simulink model "can-signal-sim"  (R2024b)
settings: Solver=VariableStepAuto  StartTime=0.0  StopTime=inf  RelTol=1e-3
undefined symbols (not defined in the file): Blinktakt, canChannel, Normal
libraries: canlib x14, canmsglib x12, simulink x6
settings Model: Creator=MBade  LastModifiedBy=MBade

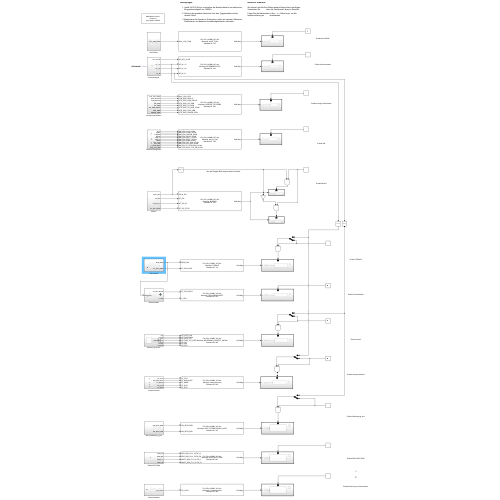
[thumbnail: Simulink's stored preview of the top-level diagram]
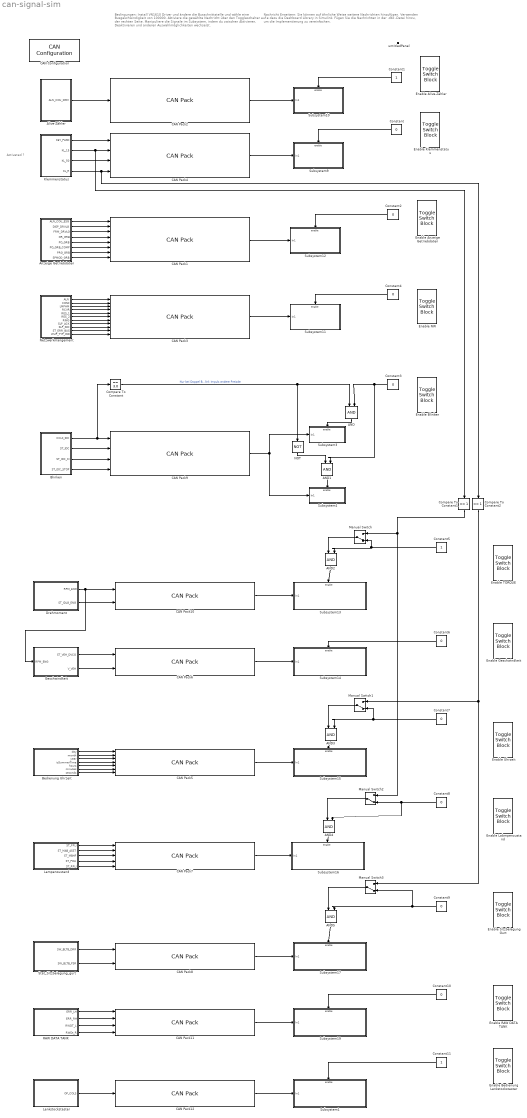
== system can-signal-sim ==
  note: Nachricht Erweitern:
      | Sie können auf ähnliche Weise weitere Nachrichten hinzufügen. Verwenden Sie dazu die Dashboard Library in Simulink.
      | Fügen Sie die Nachrichten in der .dbc -Datei hinzu, um die Implementierung zu vereinfachen.
  note: Bedingungen:
      | Install VN1610 Driver und ändere die Busschnittstelle und wähle eine Busgeschwindigkeit von 100000.
      | Aktiviere die gewählte Nachricht über den Toggleschalter auf der rechten Seite.
      | Manipuliere die Signale im Subsystem, indem du zwischen Aktivieren, Deaktivieren und anderen Auswahlmöglichkeiten wechselst.
  note: Activated ?
  AND{,1..5} (6 alike) : Logic  IconShape=distinctive  AllPortsSameDT=off  OutDataTypeStr=boolean
  Alive-Zähler : Subsystem
  Anzeige Getriebdaten : Subsystem
  Bedienung Uhrzeit : Subsystem
  Blinken : Subsystem
  CAN Configuration : canlib/CAN Configuration  BlockHandle=614.0004  Device=MathWorks Virtual 1 (Channel 1)  DeviceMenu=MathWorks Virtual 1 (Channel 1)  ObjConstructor=canChannel('MathWorks', 'Virtual 1', 1)  BusSpeed=100000  EnableBitParameters=off  AckMode=Normal
  CAN Pack1 : canmsglib/CAN Pack  CANdbFile=C:\Users\MBade\Desktop\GITHUB\Instrument-Cluster\PKW_Kombiinstruments\E9x_KOMBI_V07.dbc  MsgList=ANZEIGE_GETRIEBE  MsgName=ANZEIGE_GETRIEBE  MsgIDType=Standard (11-bit identifier)  MsgIdentifier=466  CANIDInput=off  MsgLength=6  Remote=off  ApplyMinMax=off  BusOutput=off  SignalInfo={'ALIV_COU_EGS','28','4','LE','unsigned','Standard','0','1','0','0','15';'CTR_DISP_DRVLG','40','4','LE','unsigned','Standard','0','1','0','0','15';'CTR_DISP_FRM_DRVLG','44','4','LE','unsigned','Standard','0','1','0','0','15';'CTR_DISP_GR_GRB','12','4','LE','unsigned','Standard','0','1','0','0','15';'CTR_DISP_PO_GRB','0','4','LE','unsigned','Standard','0','1','0','0','15';'CTR_DISP_PO_GRB_COMP','4','4','LE','unsigned','Standard','0','1','0','0','15';'CTR_DISP_PRG_GRB','32','4','LE','unsigned','Standard','0','1','0','0','15';'CTR_DISP_SPMOD_GRB','26','2','LE','unsigned','Standard','0','1','0','0','3'}
      settings: LibrarySourceBlock=canlib/CAN Pack  DataFormat=CANdb specified signals
  CAN Pack10 : canmsglib/CAN Pack  CANdbFile=C:\Users\MBade\MATLAB\Projects\PKW_Kombiinstruments\E9x_KOMBI_V07.dbc  MsgList=TORQUE  MsgName=TORQUE  MsgIDType=Standard (11-bit identifier)  MsgIdentifier=170  CANIDInput=off  MsgLength=8  Remote=off  ApplyMinMax=off  BusOutput=off  SignalInfo={'RPM_ENG','32','16','LE','unsigned','Standard','0','0.25','0','0','16383.75';'ST_IDLG_ENG','50','2','LE','unsigned','Standard','0','1','0','0','3'}
      settings: LibrarySourceBlock=canlib/CAN Pack  DataFormat=CANdb specified signals
  CAN Pack11 : canmsglib/CAN Pack  CANdbFile=C:\Users\MBade\MATLAB\Projects\PKW_Kombiinstruments\E9x_KOMBI_V07.dbc  MsgList=RAW_DATA_TANK  MsgName=RAW_DATA_TANK  MsgIDType=Standard (11-bit identifier)  MsgIdentifier=841  CANIDInput=off  MsgLength=5  Remote=off  ApplyMinMax=off  BusOutput=off  SignalInfo={'ERR_SEN_FLLV_FUTA_LH','32','4','LE','unsigned','Standard','0','1','0','0','15';'ERR_SEN_FLLV_FUTA_RH','36','4','LE','unsigned','Standard','0','1','0','0','15';'RWDT_SEN_FLLV_FUTA_L','0','16','LE','unsigned','Standard','0','0.1','0','0','6553.5';'RWDT_SEN_FLLV_FUTA_R','16','16','LE','unsigned','Standard','0','0.1','0','0','6553.5'}
      settings: LibrarySourceBlock=canlib/CAN Pack  DataFormat=CANdb specified signals
  CAN Pack12 : canmsglib/CAN Pack  CANdbFile=C:\Users\MBade\MATLAB\Projects\PKW_Kombiinstruments\E9x_KOMBI_V07.dbc  MsgList=Lenkstockstaster  MsgName=Lenkstockstaster  MsgIDType=Standard (11-bit identifier)  MsgIdentifier=494  CANIDInput=off  MsgLength=2  Remote=off  ApplyMinMax=off  BusOutput=off  SignalInfo={'OP_COLS','0','8','LE','unsigned','Standard','0','1','0','-Inf','Inf'}
      settings: LibrarySourceBlock=canlib/CAN Pack  DataFormat=CANdb specified signals
  CAN Pack2 : canmsglib/CAN Pack  CANdbFile=C:\Users\MBade\Desktop\GITHUB\Instrument-Cluster\PKW_Kombiinstruments\E9x_KOMBI_V07.dbc  MsgList=ALIVE_ZGM  MsgName=ALIVE_ZGM  MsgIDType=Standard (11-bit identifier)  MsgIdentifier=192  CANIDInput=off  MsgLength=2  Remote=off  ApplyMinMax=off  BusOutput=off  SignalInfo={'ALIV_COU_ZGM','0','4','LE','unsigned','Standard','0','1','0','0','15'}
      settings: LibrarySourceBlock=canlib/CAN Pack  DataFormat=CANdb specified signals
  CAN Pack3 : canmsglib/CAN Pack  CANdbFile=C:\Users\MBade\Desktop\GITHUB\Instrument-Cluster\PKW_Kombiinstruments\E9x_KOMBI_V07.dbc  MsgList=NM_K_CAN  MsgName=NM_K_CAN  MsgIDType=Standard (11-bit identifier)  MsgIdentifier=1152  CANIDInput=off  MsgLength=8  Remote=off  ApplyMinMax=off  BusOutput=off  SignalInfo={'NM_PDU_ALIV_KCAN','8','1','LE','unsigned','Standard','0','1','0','0','1';'NM_PDU_CONF_KCAN','14','1','LE','unsigned','Standard','0','1','0','0','1';'NM_PDU_LMPHM_KCAN','10','1','LE','unsigned','Standard','0','1','0','0','1';'NM_PDU_RCVR_KCAN','0','8','LE','unsigned','Standard','0','1','0','0','255';'NM_PDU_RES_1_KCAN','11','1','LE','unsigned','Standard','0','1','0','0','1';'NM_PDU_RES_2_KCAN','15','1','LE','unsigned','Standard','0','1','0','0','1';'NM_PDU_RING_KCAN','9','1','LE','unsigned','Standard','0','1','0','0','1';'NM_PDU_SLP_ACK_KCAN','13','1','LE','unsigned','Standard','0','1','0','0','1';'NM_PDU_SLP_IND_KCAN','12','1','LE','unsigned','Standard','0','1','0','0','1';'NM_PDU_ST_ERR_BUS_KCAN','24','8','LE','unsigned','Standard','0','1','0','0','255';'NM_PDU_WUP_TYP_IND_KCAN','16','2','LE','unsigned','Standard','0','1','0','0','3'}
      settings: LibrarySourceBlock=canlib/CAN Pack  DataFormat=CANdb specified signals
  CAN Pack4 : canmsglib/CAN Pack  CANdbFile=C:\Users\MBade\Desktop\GITHUB\Instrument-Cluster\PKW_Kombiinstruments\E9x_KOMBI_V07.dbc  MsgList=KLEMMENSTATUS  MsgName=KLEMMENSTATUS  MsgIDType=Standard (11-bit identifier)  MsgIdentifier=304  CANIDInput=off  MsgLength=5  Remote=off  ApplyMinMax=off  BusOutput=off  SignalInfo={'ST_KEY_PLGD','16','2','LE','unsigned','Standard','0','1','0','0','3';'ST_KL_15','2','2','LE','unsigned','Standard','0','1','0','0','3';'ST_KL_50','4','2','LE','unsigned','Standard','0','1','0','0','3';'ST_KL_R','0','2','LE','unsigned','Standard','0','1','0','0','3'}
      settings: LibrarySourceBlock=canlib/CAN Pack  DataFormat=CANdb specified signals
  CAN Pack5 : canmsglib/CAN Pack  CANdbFile=C:\Users\MBade\MATLAB\Projects\PKW_Kombiinstruments\E9x_KOMBI_V07.dbc  MsgList=BEDIENUNG_UHRZEIT_DATUM  MsgName=BEDIENUNG_UHRZEIT_DATUM  MsgIDType=Standard (11-bit identifier)  MsgIdentifier=926  CANIDInput=off  MsgLength=8  Remote=off  ApplyMinMax=off  BusOutput=off  SignalInfo={'OP_DATE_DAY','24','8','LE','unsigned','Standard','0','1','0','0','255';'OP_DATE_MON','36','4','LE','unsigned','Standard','0','1','0','0','15';'OP_DATE_YR','40','16','LE','unsigned','Standard','0','1','0','0','65535';'OP_DISP_CTI_DATE','56','4','LE','unsigned','Standard','0','1','0','0','15';'OP_HR','0','8','LE','unsigned','Standard','0','1','0','0','255';'OP_MN','8','8','LE','unsigned','Standard','0','1','0','0','255';'OP_SEC','16','8','LE','unsigned','Standard','0','1','0','0','255'}
      settings: LibrarySourceBlock=canlib/CAN Pack  DataFormat=CANdb specified signals
  CAN Pack6 : canmsglib/CAN Pack  CANdbFile=C:\Users\MBade\MATLAB\Projects\PKW_Kombiinstruments\E9x_KOMBI_V07.dbc  MsgList=GESCHWINDIGKEIT  MsgName=GESCHWINDIGKEIT  MsgIDType=Standard (11-bit identifier)  MsgIdentifier=416  CANIDInput=off  MsgLength=8  Remote=off  ApplyMinMax=off  BusOutput=off  SignalInfo={'ST_VEH_DVCO','12','3','LE','unsigned','Standard','0','1','0','0','7';'V_VEH','0','12','LE','unsigned','Standard','0','0.1','0','0','409.5'}
      settings: LibrarySourceBlock=canlib/CAN Pack  DataFormat=CANdb specified signals
  CAN Pack7 : canmsglib/CAN Pack  CANdbFile=C:\Users\MBade\MATLAB\Projects\PKW_Kombiinstruments\E9x_KOMBI_V07.dbc  MsgList=Lampenzustand  MsgName=Lampenzustand  MsgIDType=Standard (11-bit identifier)  MsgIdentifier=538  CANIDInput=off  MsgLength=3  Remote=off  ApplyMinMax=off  BusOutput=off  SignalInfo={'ST_FFLI','5','1','LE','unsigned','Standard','0','1','0','-Inf','Inf';'ST_MAB_ASST','18','2','LE','unsigned','Standard','0','1','0','-Inf','Inf';'ST_MBHF','1','1','LE','unsigned','Standard','0','1','0','-Inf','Inf';'ST_POLI','2','1','LE','unsigned','Standard','0','1','0','-Inf','Inf';'ST_RFLI','6','1','LE','unsigned','Standard','0','1','0','-Inf','Inf'}
      settings: LibrarySourceBlock=canlib/CAN Pack  DataFormat=CANdb specified signals
  CAN Pack8 : canmsglib/CAN Pack  CANdbFile=C:\Users\MBade\MATLAB\Projects\PKW_Kombiinstruments\E9x_KOMBI_V07.dbc  MsgList=STAT_SITZBELEGUNG_GURT  MsgName=STAT_SITZBELEGUNG_GURT  MsgIDType=Standard (11-bit identifier)  MsgIdentifier=762  CANIDInput=off  MsgLength=5  Remote=off  ApplyMinMax=off  BusOutput=off  SignalInfo={'SW_BLTB_DRR','28','2','LE','unsigned','Standard','0','1','0','0','3';'SW_BLTB_PSR','30','2','LE','unsigned','Standard','0','1','0','0','3'}
      settings: LibrarySourceBlock=canlib/CAN Pack  DataFormat=CANdb specified signals
  CAN Pack9 : canmsglib/CAN Pack  CANdbFile=C:\Users\MBade\MATLAB\Projects\PKW_Kombiinstruments\E9x_KOMBI_V07.dbc  MsgList=BLINKEN  MsgName=BLINKEN  MsgIDType=Standard (11-bit identifier)  MsgIdentifier=502  CANIDInput=off  MsgLength=2  Remote=off  ApplyMinMax=off  BusOutput=off  SignalInfo={'CCLK_IDC','0','4','LE','unsigned','Standard','0','1','0','0','15';'ST_IDC','4','3','LE','unsigned','Standard','0','1','0','0','7';'ST_IDC_KI','10','2','LE','unsigned','Standard','0','1','0','0','3';'ST_IDC_STOP','8','2','LE','unsigned','Standard','0','1','0','0','3'}
      settings: LibrarySourceBlock=canlib/CAN Pack  DataFormat=CANdb specified signals
  Compare To Constant : simulink/Logic and Bit Operations/Compare To Constant  relop===  const=3.0  OutDataTypeStr=boolean
  Compare To Constant1 : simulink/Logic and Bit Operations/Compare To Constant  relop===  const=1  OutDataTypeStr=boolean
  Compare To Constant2 : simulink/Logic and Bit Operations/Compare To Constant  relop===  const=1  OutDataTypeStr=boolean
  Constant{,2..4,6..10} (9 alike) : Constant  Value=0
  Constant1 : Constant
  Constant11 : Constant
  Constant5 : Constant
  Drehmoment : Subsystem
  Enable Alive-Zähler : ToggleSwitchBlock
      settings: Values={{'Off', 'On'}, [0 1]}
  Enable Anzeige Getriebdaten : ToggleSwitchBlock
      settings: Values={{'Off', 'On'}, [0 1]}
  Enable Bedienung Lenkstockstaster : ToggleSwitchBlock
      settings: Values={{'Off', 'On'}, [0 1]}
  Enable Blinken : ToggleSwitchBlock
      settings: Values={{'Off', 'On'}, [0 1]}
  Enable Geschwindkeit : ToggleSwitchBlock
      settings: Values={{'Off', 'On'}, [0 1]}
  Enable Klemmenstatus : ToggleSwitchBlock
      settings: Values={{'Off', 'On'}, [0 1]}
  Enable Labmpenzustand : ToggleSwitchBlock
      settings: Values={{'Off', 'On'}, [0 1]}
  Enable NW : ToggleSwitchBlock
      settings: Values={{'Off', 'On'}, [0 1]}
  Enable RAW DATA TANK : ToggleSwitchBlock
      settings: Values={{'Off', 'On'}, [0 1]}
  Enable Sitzbelegung Gurt : ToggleSwitchBlock
      settings: Values={{'Off', 'On'}, [0 1]}
  Enable TORQUE : ToggleSwitchBlock
      settings: Values={{'Off', 'On'}, [0 1]}
  Enable Uhrzeit : ToggleSwitchBlock
      settings: Values={{'Off', 'On'}, [0 1]}
  Geschwindkeit : Subsystem
  Klemmenstatus : Subsystem
  Lampenzustand : Subsystem
  Lenkstockstaster : Subsystem
  Manual Switch{,1..3} (4 alike) : ManualSwitch  CurrentSetting=0
  NOT : Logic  Operator=NOT  IconShape=distinctive  AllPortsSameDT=off  OutDataTypeStr=boolean
  Netzwerkmangement : Subsystem
  RAW DATA TANK : Subsystem
  Stat_Sitzbelegung_gurt : Subsystem
  Subsystem1 : Subsystem
  Subsystem10 : Subsystem
  Subsystem11 : Subsystem
  Subsystem12 : Subsystem
  Subsystem13 : Subsystem
  Subsystem14 : Subsystem
  Subsystem15 : Subsystem
  Subsystem16 : Subsystem
  Subsystem17 : Subsystem
  Subsystem19 : Subsystem
  Subsystem3 : Subsystem
  Subsystem4 : Subsystem
  Subsystem9 : Subsystem
  untitledPanel : Subsystem  Tag=HiddenForWebPanel  IsWebBlockPanel=on
  wires:
  Anzeige Getriebdaten/5(PO_GRB) -> CAN Pack1/5
  Anzeige Getriebdaten/6(PO_GRB_COMP) -> CAN Pack1/6
  Anzeige Getriebdaten/2(DISP_DRVLG) -> CAN Pack1/2
  Anzeige Getriebdaten/1(ALIV_COU_ESG) -> CAN Pack1/1
  Anzeige Getriebdaten/3(FRM_DRVLG) -> CAN Pack1/3
  Anzeige Getriebdaten/4(GR_GRB) -> CAN Pack1/4
  Anzeige Getriebdaten/8(SPMOD_GRB) -> CAN Pack1/8
  Anzeige Getriebdaten/7(PRG_GRB) -> CAN Pack1/7
  Alive-Zähler/1(ALIV_COU_ZGM) -> CAN Pack2/1
  Netzwerkmangement/5(RES_1) -> CAN Pack3/5
  Netzwerkmangement/7(RING) -> CAN Pack3/7
  Netzwerkmangement/6(RES_2) -> CAN Pack3/6
  Netzwerkmangement/4(RCVR) -> CAN Pack3/4
  Netzwerkmangement/8(SLP_ACK) -> CAN Pack3/8
  Netzwerkmangement/11(WUP_TYP_IND) -> CAN Pack3/11
  Netzwerkmangement/2(CONF) -> CAN Pack3/2
  Netzwerkmangement/9(SLP_IND) -> CAN Pack3/9
  Netzwerkmangement/10(ST_ERR_BUS) -> CAN Pack3/10
  Netzwerkmangement/1(ALIV) -> CAN Pack3/1
  Netzwerkmangement/3(LMPHM) -> CAN Pack3/3
  Klemmenstatus/1(KEY_PLGD) -> CAN Pack4/1
  Klemmenstatus/3(KL_50) -> CAN Pack4/3
  Klemmenstatus/4(KL_R) -> Compare To Constant2/1, CAN Pack4/4
  Blinken/1(CCLK_IDC) -> Compare To Constant/1, CAN Pack9/1
  Blinken/2(ST_IDC) -> CAN Pack9/2
  Blinken/3(ST_IDC_KI) -> CAN Pack9/3
  Blinken/4(ST_IDC_STOP) -> CAN Pack9/4
  Compare To Constant/1 -> AND/1, NOT/1  "Nur bei Doppel Blink Impuls andere Preiode"
  CAN Pack9/1 -> Subsystem4/1(In1), Subsystem3/1(In1)
  Drehmoment/1(RPM_ENG) -> CAN Pack10/1, Geschwindkeit/1(RPM_ENG)
  Drehmoment/2(ST_IDLG_ENG) -> CAN Pack10/2
  Geschwindkeit/1(ST_VEH_DVCO) -> CAN Pack6/1
  Geschwindkeit/2(V_VEH) -> CAN Pack6/2
  Klemmenstatus/2(KL_15) -> CAN Pack4/2, Compare To Constant1/1
  Compare To Constant1/1 -> Manual Switch2/1, Manual Switch/1
  Bedienung Uhrzeit/1(day) -> CAN Pack5/1
  Bedienung Uhrzeit/2(month) -> CAN Pack5/2
  Bedienung Uhrzeit/3(year) -> CAN Pack5/3
  Bedienung Uhrzeit/4(isSummerTime) -> CAN Pack5/4
  Bedienung Uhrzeit/5(hours) -> CAN Pack5/5
  Bedienung Uhrzeit/6(minutes) -> CAN Pack5/6
  Bedienung Uhrzeit/7(seconds) -> CAN Pack5/7
  Lampenzustand/1(ST_FFLI) -> CAN Pack7/1
  Lampenzustand/2(ST_MAB_ASST) -> CAN Pack7/2
  Lampenzustand/3(ST_MBHF) -> CAN Pack7/3
  Lampenzustand/4(ST_POLI) -> CAN Pack7/4
  Lampenzustand/5(ST_RFLI) -> CAN Pack7/5
  CAN Pack4/1 -> Subsystem9/1(In1)
  Constant/1 -> Subsystem9/Enable
  CAN Pack2/1 -> Subsystem10/1(In1)
  Constant1/1 -> Subsystem10/Enable
  CAN Pack3/1 -> Subsystem11/1(In1)
  CAN Pack1/1 -> Subsystem12/1(In1)
  Constant2/1 -> Subsystem12/Enable
  Constant4/1 -> Subsystem11/Enable
  NOT/1 -> AND1/1
  Constant3/1 -> AND/2, AND1/2
  AND1/1 -> Subsystem4/Enable
  AND/1 -> Subsystem3/Enable
  CAN Pack10/1 -> Subsystem13/1(In1)
  AND2/1 -> Subsystem13/Enable
  Constant5/1 -> AND2/2, Manual Switch/2
  Manual Switch/1 -> AND2/1
  CAN Pack6/1 -> Subsystem14/1(In1)
  Constant6/1 -> Subsystem14/Enable
  CAN Pack5/1 -> Subsystem15/1(In1)
  AND3/1 -> Subsystem15/Enable
  Constant7/1 -> AND3/2, Manual Switch1/2
  Compare To Constant2/1 -> Manual Switch1/1, Manual Switch3/1
  Manual Switch1/1 -> AND3/1
  CAN Pack7/1 -> Subsystem16/1(In1)
  AND4/1 -> Subsystem16/Enable
  Manual Switch2/1 -> AND4/1
  Constant8/1 -> Manual Switch2/2, AND4/2
  AND5/1 -> Subsystem17/Enable
  Manual Switch3/1 -> AND5/1
  Constant9/1 -> Manual Switch3/2, AND5/2
  CAN Pack8/1 -> Subsystem17/1(In1)
  Stat_Sitzbelegung_gurt/1(SW_BLTB_DRR) -> CAN Pack8/1
  Stat_Sitzbelegung_gurt/2(SW_BLTB_PSR) -> CAN Pack8/2
  CAN Pack11/1 -> Subsystem19/1(In1)
  Constant10/1 -> Subsystem19/Enable
  RAW DATA TANK/1(ERR_LH) -> CAN Pack11/1
  RAW DATA TANK/3(RWDT_L) -> CAN Pack11/3
  RAW DATA TANK/2(ERR_RH) -> CAN Pack11/2
  RAW DATA TANK/4(RWDt_R) -> CAN Pack11/4
  Constant11/1 -> Subsystem1/Enable
  CAN Pack12/1 -> Subsystem1/1(In1)
  Lenkstockstaster/1(OP_COLS) -> CAN Pack12/1

== system can-signal-sim/Alive-Zähler ==
  note: Die Versendung dieser Nachricht erfolgt zyklisch bei Bus aktiv.
  Constant : Constant  Value=15  OutDataTypeStr=uint8  SampleTime=0.2
  Counter Limited1 : simulink/Sources/Counter Limited  uplimit=14  tsamp=0.2
  Display : Display
      settings: Format=binary (Stored Integer)
  Manual Switch : ManualSwitch
  Scope : Scope
  ALIV_COU_ZGM : Outport
  wires:
  Manual Switch/1 -> Display/1, ALIV_COU_ZGM/1, Scope/1  "ALIV_COU_ZGM"
  Constant/1 -> Manual Switch/2  "Signal ungültig"
  Counter Limited1/1 -> Manual Switch/1

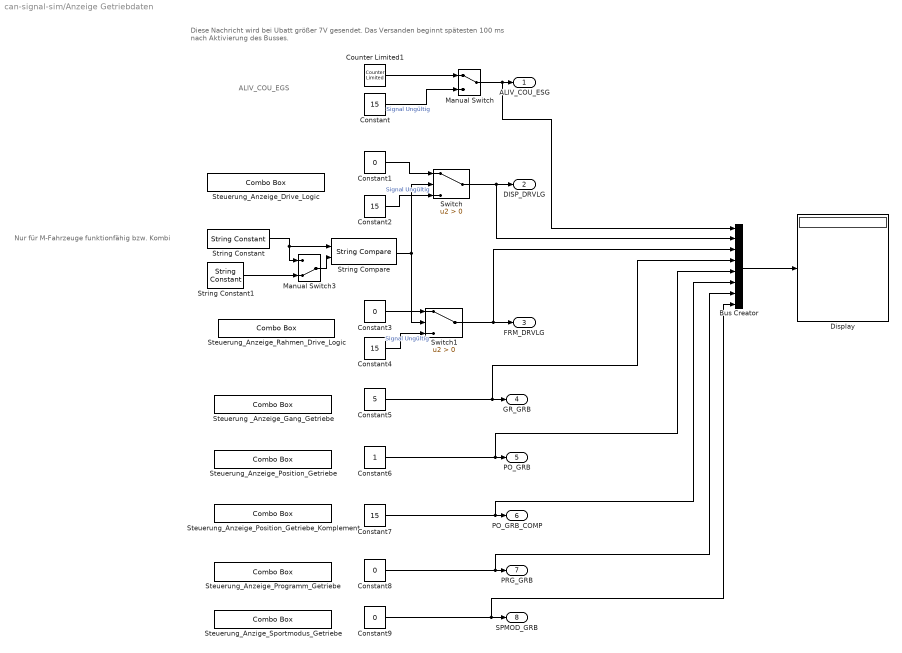
== system can-signal-sim/Anzeige Getriebdaten ==
  note: Nur für M-Fahrzeuge funktionfähig bzw. Kombi
  note: ALIV_COU_EGS
  note: Diese Nachricht wird bei Ubatt größer 7V gesendet. Das Versanden beginnt spätesten 100 ms nach Aktivierung des Busses.
  Bus Creator : BusCreator  Inputs=8
  Constant{,2,4,7} (4 alike) : Constant  Value=15  SampleTime=0.2
  Constant{1,3,8..9} (4 alike) : Constant  Value=0  SampleTime=0.2
  Constant5 : Constant  Value=5  SampleTime=0.2
  Constant6 : Constant  SampleTime=0.2
  Counter Limited1 : simulink/Sources/Counter Limited  uplimit=14  tsamp=0.2
  Display : Display
      settings: Format=binary (Stored Integer)
  Manual Switch : ManualSwitch
  Manual Switch3 : ManualSwitch  CurrentSetting=0
  Steuerung _Anzeige_Gang_Getriebe : ComboBox  LabelPosition=Hide  SelectedLabel=1.Gang
      settings: Values={{'Dunkelschaltung', '1.Gang', '2.Gang', '3.Gang', '4.Gang', '5.Gang', '6.Gang', '7.Gang', '8.Gang', 'Signal ungültig'}, [0 5 6 7 8 9 10 11 12 15]}
  Steuerung_Anzeige_Drive_Logic : ComboBox  LabelPosition=Hide  SelectedLabel=Dunkelschaltung
      settings: Values={{'Dunkelschaltung', '1', '2', '3', '4', '5', '6', 'Signal ungültig'}, [0 1 2 3 4 5 6 15]}
  Steuerung_Anzeige_Position_Getriebe : ComboBox  LabelPosition=Hide  SelectedLabel=P
      settings: Values={{'Dunkelschaltung', 'P', 'R', 'P_30sec', 'N', 'N_30,5min', 'N-5min', 'D', 'Signal ungültig'}, [0 1 2 3 4 6 7 8 15]}
  Steuerung_Anzeige_Position_Getriebe_Komplement : ComboBox  LabelPosition=Hide  SelectedLabel=Dunkelschaltung
      settings: Values={{'Dunkelschaltung', 'P', 'R', 'P_30sec', 'N', 'N_30,5min', 'N_5min', 'D', 'Signal ungültig'}, [15 14 13 12 11 9 8 7 0]}
  Steuerung_Anzeige_Programm_Getriebe : ComboBox  LabelPosition=Hide  SelectedLabel=Dunkelschaltung
      settings: Values={{'Dunkelschaltung', 'S-Programm', 'M-Programm', 'L-Programm', 'C-Programm', 'Signal ungültig'}, [0 1 2 4 8 15]}
  Steuerung_Anzeige_Rahmen_Drive_Logic : ComboBox  LabelPosition=Hide  SelectedLabel=Dunkelschaltung
      settings: Values={{'Dunkelschaltung', 'An, 5 Segmente', 'An, 6 Segmente', 'Signal ungültig'}, [0 5 6 15]}
  Steuerung_Anzige_Sportmodus_Getriebe : ComboBox  LabelPosition=Hide  SelectedLabel=Normalmodus
      settings: Values={{'Normalmodus', 'Sportmodus', 'Signal ungültig'}, [0 1 3]}
  String Compare : StringCompare
  String Constant : StringConstant  String="\"M_Fahrzeugen\""
  String Constant1 : StringConstant  String="\"anders\""
  Switch : Switch  Criteria=u2 > Threshold  SaturateOnIntegerOverflow=off  InputSameDT=off
  Switch1 : Switch  Criteria=u2 > Threshold  SaturateOnIntegerOverflow=off  InputSameDT=off
  ALIV_COU_ESG : Outport
  DISP_DRVLG : Outport  Port=2
  FRM_DRVLG : Outport  Port=3
  GR_GRB : Outport  Port=4
  PO_GRB : Outport  Port=5
  PO_GRB_COMP : Outport  Port=6
  PRG_GRB : Outport  Port=7
  SPMOD_GRB : Outport  Port=8
  wires:
  Counter Limited1/1 -> Manual Switch/1
  Manual Switch/1 -> ALIV_COU_ESG/1, Bus Creator/1
  Switch1/1 -> Bus Creator/3, FRM_DRVLG/1
  Constant/1 -> Manual Switch/2  "Signal Ungültig"
  Constant5/1 -> Bus Creator/4, GR_GRB/1
  Constant6/1 -> Bus Creator/5, PO_GRB/1
  Constant7/1 -> Bus Creator/6, PO_GRB_COMP/1
  Constant8/1 -> Bus Creator/7, PRG_GRB/1
  Constant9/1 -> Bus Creator/8, SPMOD_GRB/1
  String Constant/1 -> Manual Switch3/1, String Compare/1
  String Constant1/1 -> Manual Switch3/2
  Manual Switch3/1 -> String Compare/2
  String Compare/1 -> Switch/2, Switch1/2
  Constant1/1 -> Switch/1
  Constant2/1 -> Switch/3  "Signal Ungültig"
  Switch/1 -> Bus Creator/2, DISP_DRVLG/1
  Constant4/1 -> Switch1/3  "Signal Ungültig"
  Constant3/1 -> Switch1/1
  Bus Creator/1 -> Display/1

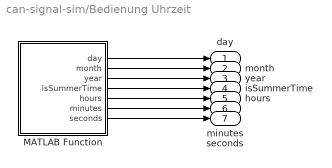
== system can-signal-sim/Bedienung Uhrzeit ==
  MATLAB Function : MATLAB Function  TreatAsAtomicUnit=on
  day : Outport
  month : Outport  Port=2
  year : Outport  Port=3
  isSummerTime : Outport  Port=4
  hours : Outport  Port=5
  minutes : Outport  Port=6
  seconds : Outport  Port=7
  wires:
  MATLAB Function/4(isSummerTime) -> isSummerTime/1
  MATLAB Function/6(minutes) -> minutes/1
  MATLAB Function/5(hours) -> hours/1
  MATLAB Function/7(seconds) -> seconds/1
  MATLAB Function/3(year) -> year/1
  MATLAB Function/2(month) -> month/1
  MATLAB Function/1(day) -> day/1

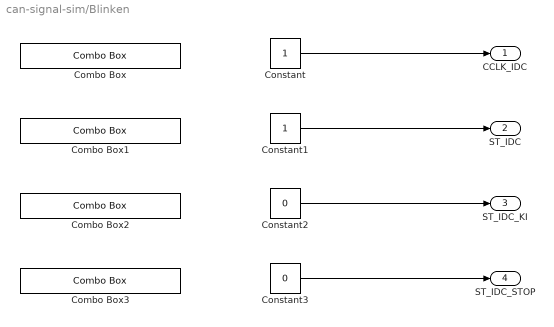
== system can-signal-sim/Blinken ==
  Combo Box : ComboBox  LabelPosition=Hide  SelectedLabel=Normal-Blinktakt
      settings: Values={{'Nicht blinken', 'Normal-Blinktakt', 'Defekt-Blinktakt', 'Doppel-Blink-Impuls', 'Signal ungültig'}, [0 1 2 3 15]}
  Combo Box1 : ComboBox  LabelPosition=Hide  SelectedLabel=Blinker link Ein
      settings: Values={{'Beide Blinker AUS', 'Blinker link Ein', 'Blinker rechts Ein', 'Beide Blinker Ein', 'Signal ungültig'}, [0 1 2 3 7]}
  Combo Box2 : ComboBox  LabelPosition=Hide  SelectedLabel=Blinktakt läuft weiter
      settings: Values={{'Blinktakt läuft weiter', 'Synchronisation', 'Neuen Blinktakt starten', 'Signal ungültig'}, [0 1 2 3]}
  Combo Box3 : ComboBox  LabelPosition=Hide  SelectedLabel=Blinkerkontroll-Lampen im Kombi signalisieren
      settings: Values={{'Blinkerkontroll-Lampen im Kombi signalisieren', 'Blinkerkontroll-Lampen im verdecktes Blinken', 'Signal ungültig'}, [0 1 3]}
  Constant : Constant
  Constant1 : Constant
  Constant2 : Constant  Value=0
  Constant3 : Constant  Value=0
  CCLK_IDC : Outport
  ST_IDC : Outport  Port=2
  ST_IDC_KI : Outport  Port=3
  ST_IDC_STOP : Outport  Port=4
  wires:
  Constant/1 -> CCLK_IDC/1
  Constant1/1 -> ST_IDC/1
  Constant2/1 -> ST_IDC_KI/1
  Constant3/1 -> ST_IDC_STOP/1

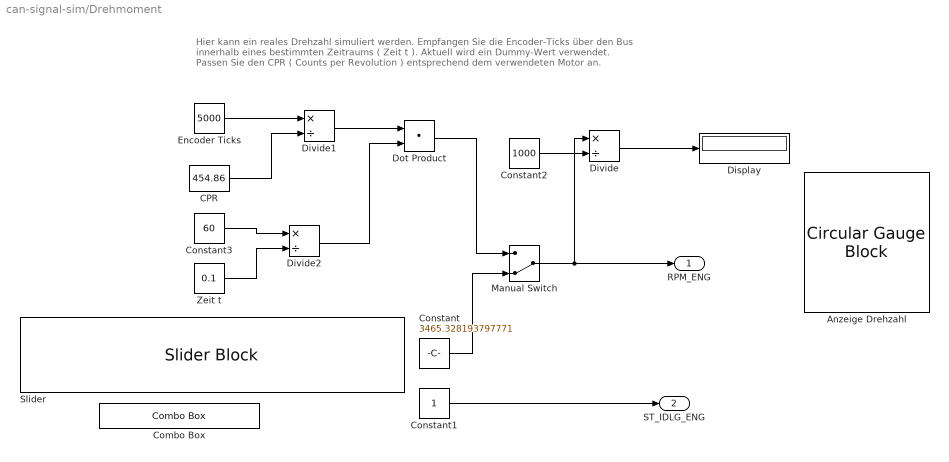
== system can-signal-sim/Drehmoment ==
  note: Hier kann ein reales Drehzahl simuliert werden.
      | Empfangen Sie die Encoder-Ticks über den Bus innerhalb eines bestimmten Zeitraums ( Zeit t ).
      | Aktuell wird ein Dummy-Wert verwendet.
      | Passen Sie den CPR ( Counts per Revolution ) entsprechend dem verwendeten Motor an.
  Anzeige Drehzahl : CircularGaugeBlock  ScaleMax=6  TickInterval=1
  CPR : Constant  Value=454.86
  Combo Box : ComboBox  LabelPosition=Hide  SelectedLabel=Motor nicht im Leerlauf
      settings: Values={{'Leerlauf', 'Motor nicht im Leerlauf', 'Label3'}, [0 1 3]}
  Constant : Constant  Value=3465.328193797771  OutMax=[16383.75]
  Constant1 : Constant
  Constant2 : Constant  Value=1000
  Constant3 : Constant  Value=60
  Display : Display
  Divide : Product  Inputs=*/
  Divide1 : Product  Inputs=*/
  Divide2 : Product  Inputs=*/
  Dot Product : DotProduct  OutDataTypeStr=Inherit: Inherit via internal rule
  Encoder Ticks : Constant  Value=5000
  Manual Switch : ManualSwitch  CurrentSetting=0
  Slider : SliderBlock  ScaleMax=16383.75
  Zeit t : Constant  Value=0.1
  RPM_ENG : Outport
  ST_IDLG_ENG : Outport  Port=2
  wires:
  Constant1/1 -> ST_IDLG_ENG/1
  Constant/1 -> Manual Switch/2
  Manual Switch/1 -> RPM_ENG/1, Divide/1
  Constant2/1 -> Divide/2
  Encoder Ticks/1 -> Divide1/1
  CPR/1 -> Divide1/2
  Constant3/1 -> Divide2/1
  Divide2/1 -> Dot Product/2
  Divide1/1 -> Dot Product/1
  Zeit t/1 -> Divide2/2
  Dot Product/1 -> Manual Switch/1
  Divide/1 -> Display/1

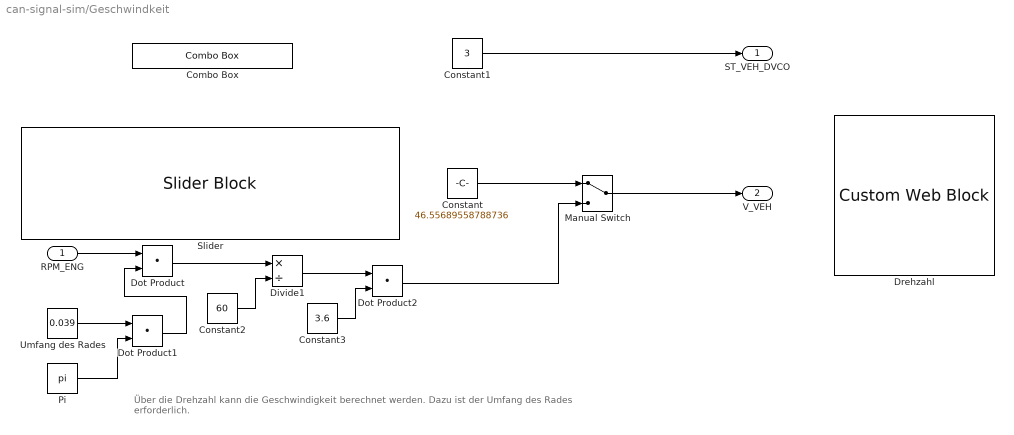
== system can-signal-sim/Geschwindkeit ==
  note: Über die Drehzahl kann die Geschwindigkeit berechnet werden. Dazu ist der Umfang des Rades erforderlich.
  RPM_ENG : Inport
  Combo Box : ComboBox  LabelPosition=Hide  SelectedLabel=Fahrzeug fährt
      settings: Values={{'Fahrzeugsteht', 'Fahrzeug fährt vorwärts', 'Fahrzeug fährt rückwärts', 'Fahrzeug fährt', 'Signal ungültig'}, [0 1 2 3 7]}
  Constant : Constant  Value=46.55689558788736  OutMax=[409.5]
  Constant1 : Constant  Value=3
  Constant2 : Constant  Value=60
  Constant3 : Constant  Value=3.6
  Divide1 : Product  Inputs=*/
  Dot Product : DotProduct  OutDataTypeStr=Inherit: Inherit via internal rule
  Dot Product1 : DotProduct  OutDataTypeStr=Inherit: Inherit via internal rule
  Dot Product2 : DotProduct  OutDataTypeStr=Inherit: Inherit via internal rule
  Drehzahl : CustomWebBlock  LabelPosition=Hide  ShowInitialText=on  Configuration="{\"components\":[{\"name\":\"CircularScaleComponent\",\"settings\":{\"bounds\":{\"max\":320,\"min\":0,\"tickInterval\":\"auto\"},\"direction\":\"cw\",\"flipLimits\":0,\"innerRadius\":0.75,\"internalTickHeightScaleFactor\":1,\"labelColor\":[255,255,200],\"labelFont\":{\"font\":\"Arial\",\"fontSize\":12},\"labelRadius\":0.528,\"labelTransparency\":1,\"minorTickHeightScaleFactor\":0.2,\"needleImage\":{\"size\":[200,50],\"src\":\"data:image\\/svg+xml;base64,PD94bWwgdmVyc2lvbj0iMS4wIiBlbmNvZGluZz0idXRmLTgiPz4KPCEtLSBHZW5lcmF0b3I6IEFkb2JlIElsbHVzdHJhdG9yIDI0LjEuMiwgU1ZHIEV4cG9ydCBQbHVnLUluIC4gU1ZHIFZlcnNpb246IDYuMDAgQnVpbGQgMCkgIC0tPgo8c3ZnIHZlcnNpb249IjEuMSIgaWQ9IkxheWVyXzEiIHhtbG5zPSJodHRwOi8vd3d3LnczLm9yZy8yMDAwL3N2ZyIgeG1sbnM6eGxpbms9Imh0dHA6Ly93d3cudzMub3JnLzE5OTkveGxpbmsiIHg9IjBweCIgeT0iMHB4IgoJIHZpZXdCb3g9IjAgMCAyMDAgNTAiIHN0eWxlPSJlbmFibGUtYmFja2dyb3VuZDpuZXcgMCAwIDIwMCA1MDsiIHhtbDpzcGFjZT0icHJlc2VydmUiPgo8c3R5bGUgdHlwZT0idGV4dC9jc3MiPgoJLnN0MHtmaWxsOiNFQzIxMjc7fQo8L3N0eWxlPgo8cGF0aCBjbGFzcz0ic3QwIiBkPSJNMTYyLjgsMTMuN0MxNjksNC40LDE4MS43LDEuOSwxOTEsOC4xczExLjgsMTguOSw1LjYsMjguMnMtMTguOSwxMS44LTI4LjIsNS42bDAsMAoJQzE1OS4xLDM1LjYsMTU2LjYsMjMsMTYyLjgsMTMuN0wxNjIuOCwxMy43eiBNMTY1LjgsMTUuOGMtNS4xLDcuNi0zLjEsMTcuOSw0LjYsMjNjNy42LDUuMSwxNy45LDMuMSwyMy00LjYKCWM1LjEtNy42LDMuMS0xNy45LTQuNi0yM2wwLDBDMTgxLjIsNi4yLDE3MC45LDguMiwxNjUuOCwxNS44eiIvPgo8cGF0aCBjbGFzcz0ic3QwIiBkPSJNMC40LDI1Ljl2LTMuM2wxNTktMi41Yy0wLjcsMi42LTAuNyw1LjIsMCw3LjhMMC40LDI1Ljl6Ii8+CjxjaXJjbGUgY2xhc3M9InN0MCIgY3g9IjE3OS42IiBjeT0iMjQiIHI9IjAuNyIvPgo8L3N2Zz4K\"},\"needleOffset\":[0.18464878250906522,0],\"needleOrientation\":-45,\"needleRotation\":180,\"needleSize\":{\"height\":0.11741692305346914,\"width\":0.46108337545091255},\"outerRadius\":0.9,\"position\":[0.05,0.05,0.9,0.9],\"referencePoint\":\"auto\",\"scaleAngle\":270,\"scaleAngleOffset\":135,\"scaleColors\":[],\"scaleColorsSize\":0.2,\"scaleDirection\":\"CW\",\"scalePosition\":[0,0,1,1],\"showLabels\":1,\"showMinorTicks\":1,\"showSpanLine\":1,\"showTicks\":1,\"tickColor\":[252,252,197],\"tickTransparency\":1,\"valueBarColor\":[0,114,189],\"valueBarPosition\":[0,0,1,1],\"valueBarSize\":0.2,\"valueBarTransparency\":1}},{\"name\":\"BackgroundImageComponent\",\"settings\":{\"image\":{\"size\":[500,500],\"src\":\"data:image\\/svg+xml;base64,PD94bWwgdmVyc2lvbj0iMS4wIiBlbmNvZGluZz0iVVRGLTgiIHN0YW5kYWxvbmU9Im5vIj8+CjxzdmcKICAgeG1sbnM6ZGM9Imh0dHA6Ly9wdXJsLm9yZy9kYy9lbGVtZW50cy8xLjEvIgogICB4bWxuczpjYz0iaHR0cDovL2NyZWF0aXZlY29tbW9ucy5vcmcvbnMjIgogICB4bWxuczpyZGY9Imh0dHA6Ly93d3cudzMub3JnLzE5OTkvMDIvMjItcmRmLXN5bnRheC1ucyMiCiAgIHhtbG5zOnN2Zz0iaHR0cDovL3d3dy53My5vcmcvMjAwMC9zdmciCiAgIHhtbG5zPSJodHRwOi8vd3d3LnczLm9yZy8yMDAwL3N2ZyIKICAgeG1sbnM6 ...(+9964 chars)\"},\"position\":[0,0,1,1],\"scaleMode\":\"0\"}},{\"name\":\"ForegroundImageComponent\",\"settings\":{\"image\":{\"size\":[0,0],\"src\":\"default\",\"srcOrientation\":[]},\"isForeground\":1,\"position\":[0,0,1,1],\"scaleMode\":\"0\"}}],\"settings\":{\"BindingType\":\"signal\",\"aspectRatio\":1.032258064516129,\"backgroundColor\":[0,0,0,\"1\"],\"backgroundOffset\":1,\"backgroundOpacity\":1,\"direction\":\"cw\",\"fixedAspectRatio\":\"on\",\"flipLimits\":0,\"orientation\":\"horizontal\",\"showBackgroundColor\":false,\"value\":0,\"version\":\"R2023a\"},\"type\":\"CircularGauge\"}"
  Manual Switch : ManualSwitch
  Pi : Constant  Value=pi  OutDataTypeStr=Inherit: Inherit via back propagation
  Slider : SliderBlock  ScaleMax=409.5
  Umfang des Rades : Constant  Value=0.039
  ST_VEH_DVCO : Outport
  V_VEH : Outport  Port=2
  wires:
  Constant/1 -> Manual Switch/1
  RPM_ENG/1 -> Dot Product/1
  Pi/1 -> Dot Product1/2
  Umfang des Rades/1 -> Dot Product1/1
  Dot Product1/1 -> Dot Product/2
  Dot Product/1 -> Divide1/1
  Constant2/1 -> Divide1/2
  Divide1/1 -> Dot Product2/1
  Constant3/1 -> Dot Product2/2
  Dot Product2/1 -> Manual Switch/2
  Manual Switch/1 -> V_VEH/1
  Constant1/1 -> ST_VEH_DVCO/1

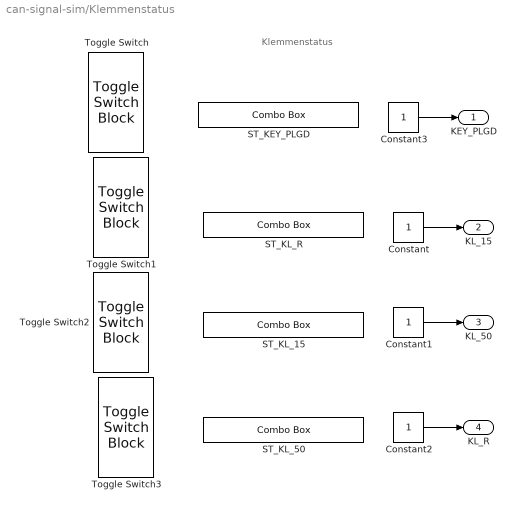
== system can-signal-sim/Klemmenstatus ==
  note: Klemmenstatus
  Constant : Constant  SampleTime=0.1
  Constant1 : Constant  SampleTime=0.1
  Constant2 : Constant  SampleTime=0.1
  Constant3 : Constant
  ST_KEY_PLGD : ComboBox  LabelPosition=Hide  SelectedLabel=Schlüssel steckt im ZAS
      settings: Values={{'Kein Schlüssel im ZAS', 'Schlüssel steckt im ZAS', 'Signal unplausibel', 'Signal ungültig'}, [0 1 2 3]}
  ST_KL_15 : ComboBox  LabelPosition=Hide  SelectedLabel=Klemme 15 EIN
      settings: Values={{'Klemme 15 AUS', 'Klemme 15 EIN', 'Reserviert', 'Signal ungültig'}, [0 1 2 3]}
  ST_KL_50 : ComboBox  LabelPosition=Hide  SelectedLabel=Klemme 50 EIN
      settings: Values={{'Klemme 50 AUS', 'Klemme 50 EIN', 'Anlassstrart-Wunsch', 'Signal ungültig'}, [0 1 2 3]}
  ST_KL_R : ComboBox  LabelPosition=Hide  SelectedLabel=Klemme R EIN
      settings: Values={{'Klemme R AUS', 'Klemme R EIN', 'Reserviert', 'Signal ungültig'}, [0 1 2 3]}
  Toggle Switch{,1..3} (4 alike) : ToggleSwitchBlock
      settings: Values={{'Off', 'On'}, [0 1]}
  KEY_PLGD : Outport
  KL_15 : Outport  Port=2
  KL_50 : Outport  Port=3
  KL_R : Outport  Port=4
  wires:
  Constant1/1 -> KL_50/1
  Constant3/1 -> KEY_PLGD/1
  Constant2/1 -> KL_R/1
  Constant/1 -> KL_15/1

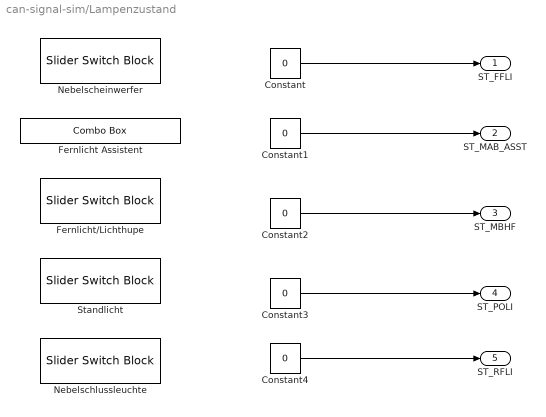
== system can-signal-sim/Lampenzustand ==
  Constant{,1..4} (5 alike) : Constant  Value=0
  Fernlicht Assistent : ComboBox  LabelPosition=Hide  SelectedLabel=AUS
      settings: Values={{'AUS', 'EIN', 'Signal ungültig'}, [0 1 3]}
  Fernlicht/Lichthupe : SliderSwitchBlock
      settings: Values={{'Off', 'On'}, [0 1]}
  Nebelscheinwerfer : SliderSwitchBlock
      settings: Values={{'Off', 'On'}, [0 1]}
  Nebelschlussleuchte : SliderSwitchBlock
      settings: Values={{'Off', 'On'}, [0 1]}
  Standlicht : SliderSwitchBlock
      settings: Values={{'Off', 'On'}, [0 1]}
  ST_FFLI : Outport
  ST_MAB_ASST : Outport  Port=2
  ST_MBHF : Outport  Port=3
  ST_POLI : Outport  Port=4
  ST_RFLI : Outport  Port=5
  wires:
  Constant/1 -> ST_FFLI/1
  Constant1/1 -> ST_MAB_ASST/1
  Constant2/1 -> ST_MBHF/1
  Constant3/1 -> ST_POLI/1
  Constant4/1 -> ST_RFLI/1

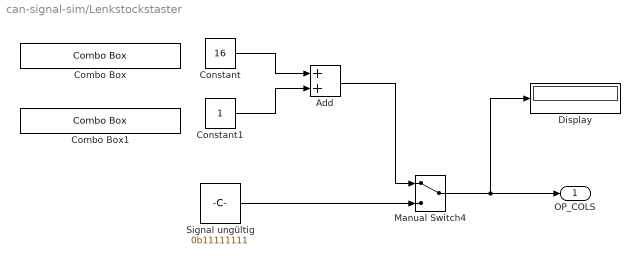
== system can-signal-sim/Lenkstockstaster ==
  Add : Sum
  Combo Box : ComboBox  LabelPosition=Hide  SelectedLabel=Tippen nach vorne
      settings: Values={{'Keine Aktion', 'Tippen nach vorne', 'Tippen nach hinten', 'Axial Tippen 1', 'Axial Tippen 2'}, [0 16 32 64 128]}
  Combo Box1 : ComboBox  LabelPosition=Hide  SelectedLabel=Tippen nach oben
      settings: Values={{'Keine Aktion', 'Tippen nach oben', 'Überdrücken nach oben', 'Überdrücken nach unten', 'Tippen nach unten'}, [0 1 2 8 4]}
  Constant : Constant  Value=16
  Constant1 : Constant
  Display : Display
      settings: Format=binary (Stored Integer)
  Manual Switch4 : ManualSwitch
  Signal ungültig : Constant  Value=0b11111111
  OP_COLS : Outport
  wires:
  Manual Switch4/1 -> OP_COLS/1, Display/1
  Constant/1 -> Add/1
  Add/1 -> Manual Switch4/1
  Signal ungültig/1 -> Manual Switch4/2
  Constant1/1 -> Add/2

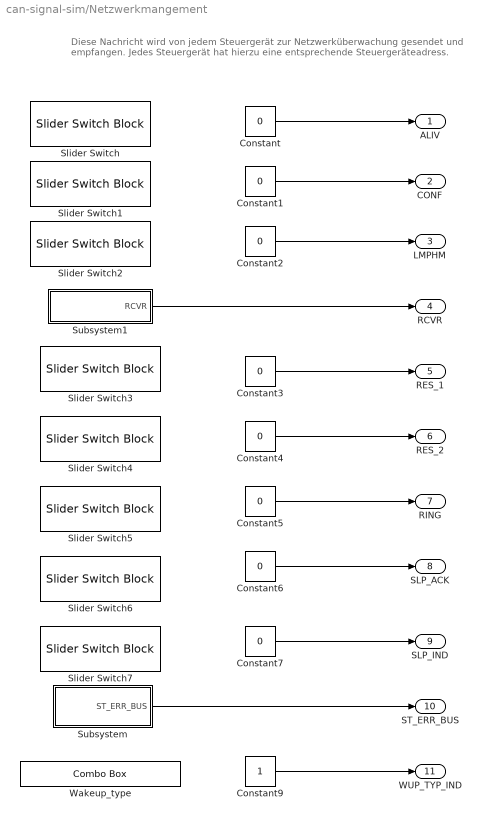
== system can-signal-sim/Netzwerkmangement ==
  note: Diese Nachricht wird von jedem Steuergerät zur Netzwerküberwachung gesendet und empfangen. Jedes Steuergerät hat hierzu eine entsprechende Steuergeräteadress.
  Constant{,1..7} (8 alike) : Constant  Value=0
  Constant9 : Constant
  Slider Switch{,1..7} (8 alike) : SliderSwitchBlock
      settings: Values={{'Off', 'On'}, [0 1]}
  Subsystem : Subsystem
  Subsystem1 : Subsystem
  Wakeup_type : ComboBox  LabelPosition=Hide  SelectedLabel=Ich habe geweckt
      settings: Values={{'Unbekannt', 'Ich habe geweckt', 'ich wurde geweckt', 'Signal ungültig'}, [0 1 2 3]}
  ALIV : Outport
  CONF : Outport  Port=2
  LMPHM : Outport  Port=3
  RCVR : Outport  Port=4
  RES_1 : Outport  Port=5
  RES_2 : Outport  Port=6
  RING : Outport  Port=7
  SLP_ACK : Outport  Port=8
  SLP_IND : Outport  Port=9
  ST_ERR_BUS : Outport  Port=10
  WUP_TYP_IND : Outport  Port=11
  wires:
  Constant4/1 -> RES_2/1
  Constant7/1 -> SLP_IND/1
  Constant1/1 -> CONF/1
  Constant2/1 -> LMPHM/1
  Constant6/1 -> SLP_ACK/1
  Subsystem/1(ST_ERR_BUS) -> ST_ERR_BUS/1
  Constant/1 -> ALIV/1
  Subsystem1/1(RCVR) -> RCVR/1
  Constant9/1 -> WUP_TYP_IND/1
  Constant5/1 -> RING/1
  Constant3/1 -> RES_1/1

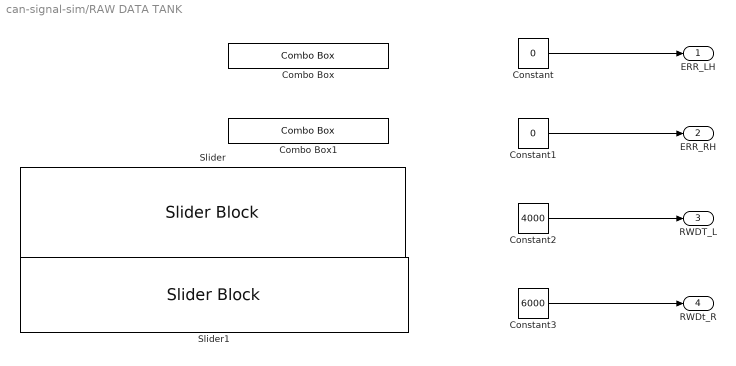
== system can-signal-sim/RAW DATA TANK ==
  Combo Box : ComboBox  LabelPosition=Hide  SelectedLabel=Sensor in Ordnung
      settings: Values={{'Sensor in Ordnung', 'Kurzschluss gegen Masse', 'Kurzschluss gegen Ubatt', 'Leitungsunterbrechung', 'Plausibilitätfehler, wert zu klein', 'Plausibilitätfehler, wert zu groß', 'Werte unterhalb Wertbereich', 'Werte oberhalb Wertbereich', 'Signal ungültig'}, [0 1 2 3 4 5 6 7 15]}
  Combo Box1 : ComboBox  LabelPosition=Hide  SelectedLabel=Sensor in Ordnung
      settings: Values={{'Sensor in Ordnung', 'Kurzschluss gegen Masse', 'Kurzschluss gegen Ubatt', 'Leitungsunterbrechung', 'Plausibilitätfehler, wert zu klein', 'Plausibilitätfehler, wert zu groß', 'Werte unterhalb Wertbereich', 'Werte oberhalb Wertbereich', 'Signal ungültig'}, [0 1 2 3 4 5 6 7 15]}
  Constant : Constant  Value=0
  Constant1 : Constant  Value=0
  Constant2 : Constant  Value=4000
  Constant3 : Constant  Value=6000
  Slider : SliderBlock  ScaleMax=6553.5  TickInterval=1000
  Slider1 : SliderBlock  ScaleMax=6553.5  TickInterval=1000
  ERR_LH : Outport
  ERR_RH : Outport  Port=2
  RWDT_L : Outport  Port=3
  RWDt_R : Outport  Port=4
  wires:
  Constant/1 -> ERR_LH/1
  Constant1/1 -> ERR_RH/1
  Constant2/1 -> RWDT_L/1
  Constant3/1 -> RWDt_R/1

== system can-signal-sim/Stat_Sitzbelegung_gurt ==
  Constant : Constant  Value=0
  Constant1 : Constant
  Schalter_Gurtschloß_BFH : ComboBox  LabelPosition=Hide  SelectedLabel=Gurt angelegt
      settings: Values={{'Gurt nicht angelegt', 'Gurt angelegt', 'Signal angelegt'}, [0 1 3]}
  Schalter_Gurtschloß_FAH : ComboBox  LabelPosition=Hide  SelectedLabel=Gurt nicht angelegt
      settings: Values={{'Gurt nicht angelegt', 'Gurt angelegt', 'Signal angelegt'}, [0 1 3]}
  SW_BLTB_DRR : Outport
  SW_BLTB_PSR : Outport  Port=2
  wires:
  Constant/1 -> SW_BLTB_DRR/1
  Constant1/1 -> SW_BLTB_PSR/1

== system can-signal-sim/Subsystem1 ==
  In1 : Inport
  Enable : EnablePort
  CAN Transmit : canlib/CAN Transmit  BlockHandle=1203.0001  Device=MathWorks Virtual 1 (Channel 1)  DeviceMenu=MathWorks Virtual 1 (Channel 1)  ObjConstructor=canChannel('MathWorks', 'Virtual 1', 1)  EnableEventTransmit=on  EnablePeriodicTransmit=on  MessagePeriod=0.1
  wires:
  In1/1 -> CAN Transmit/1

== system can-signal-sim/Subsystem10 ==
  In1 : Inport
  Enable : EnablePort
  CAN Transmit2 : canlib/CAN Transmit  BlockHandle=1212.0001  Device=MathWorks Virtual 1 (Channel 1)  DeviceMenu=MathWorks Virtual 1 (Channel 1)  ObjConstructor=canChannel('MathWorks', 'Virtual 1', 1)  EnableEventTransmit=off  EnablePeriodicTransmit=on  MessagePeriod=0.200
  wires:
  In1/1 -> CAN Transmit2/1

== system can-signal-sim/Subsystem11 ==
  In1 : Inport
  Enable : EnablePort
  CAN Transmit3 : canlib/CAN Transmit  BlockHandle=1221.0001  Device=MathWorks Virtual 1 (Channel 1)  DeviceMenu=MathWorks Virtual 1 (Channel 1)  ObjConstructor=canChannel('MathWorks', 'Virtual 1', 1)  EnableEventTransmit=off  EnablePeriodicTransmit=on  MessagePeriod=0.100
  wires:
  In1/1 -> CAN Transmit3/1

== system can-signal-sim/Subsystem12 ==
  In1 : Inport
  Enable : EnablePort
  CAN Transmit : canlib/CAN Transmit  BlockHandle=1230.0001  Device=MathWorks Virtual 1 (Channel 1)  DeviceMenu=MathWorks Virtual 1 (Channel 1)  ObjConstructor=canChannel('MathWorks', 'Virtual 1', 1)  EnableEventTransmit=off  EnablePeriodicTransmit=on  MessagePeriod=0.200
  wires:
  In1/1 -> CAN Transmit/1

== system can-signal-sim/Subsystem13 ==
  In1 : Inport
  Enable : EnablePort
  CAN Transmit9 : canlib/CAN Transmit  BlockHandle=1239.0001  Device=MathWorks Virtual 1 (Channel 1)  DeviceMenu=MathWorks Virtual 1 (Channel 1)  ObjConstructor=canChannel('MathWorks', 'Virtual 1', 1)  EnableEventTransmit=off  EnablePeriodicTransmit=on  MessagePeriod=0.100
  wires:
  In1/1 -> CAN Transmit9/1

== system can-signal-sim/Subsystem14 ==
  In1 : Inport
  Enable : EnablePort
  CAN Transmit1 : canlib/CAN Transmit  BlockHandle=1248.0001  Device=MathWorks Virtual 1 (Channel 1)  DeviceMenu=MathWorks Virtual 1 (Channel 1)  ObjConstructor=canChannel('MathWorks', 'Virtual 1', 1)  EnableEventTransmit=off  EnablePeriodicTransmit=on  MessagePeriod=0.100
  wires:
  In1/1 -> CAN Transmit1/1

== system can-signal-sim/Subsystem15 ==
  In1 : Inport
  Enable : EnablePort
  CAN Transmit4 : canlib/CAN Transmit  BlockHandle=1257.0001  Device=MathWorks Virtual 1 (Channel 1)  DeviceMenu=MathWorks Virtual 1 (Channel 1)  ObjConstructor=canChannel('MathWorks', 'Virtual 1', 1)  EnableEventTransmit=on  EnablePeriodicTransmit=on  MessagePeriod=0.100
  wires:
  In1/1 -> CAN Transmit4/1

== system can-signal-sim/Subsystem16 ==
  In1 : Inport
  Enable : EnablePort
  CAN Transmit5 : canlib/CAN Transmit  BlockHandle=1266.0001  Device=MathWorks Virtual 1 (Channel 1)  DeviceMenu=MathWorks Virtual 1 (Channel 1)  ObjConstructor=canChannel('MathWorks', 'Virtual 1', 1)  EnableEventTransmit=off  EnablePeriodicTransmit=on  MessagePeriod=5
  wires:
  In1/1 -> CAN Transmit5/1

== system can-signal-sim/Subsystem17 ==
  In1 : Inport
  Enable : EnablePort
  CAN Transmit : canlib/CAN Transmit  BlockHandle=1275.0001  Device=MathWorks Virtual 1 (Channel 1)  DeviceMenu=MathWorks Virtual 1 (Channel 1)  ObjConstructor=canChannel('MathWorks', 'Virtual 1', 1)  EnableEventTransmit=on  EnablePeriodicTransmit=on  MessagePeriod=5.000
  wires:
  In1/1 -> CAN Transmit/1

== system can-signal-sim/Subsystem19 ==
  In1 : Inport
  Enable : EnablePort
  CAN Transmit : canlib/CAN Transmit  BlockHandle=1284.0001  Device=MathWorks Virtual 1 (Channel 1)  DeviceMenu=MathWorks Virtual 1 (Channel 1)  ObjConstructor=canChannel('MathWorks', 'Virtual 1', 1)  EnableEventTransmit=on  EnablePeriodicTransmit=on  MessagePeriod=0.2
  wires:
  In1/1 -> CAN Transmit/1

== system can-signal-sim/Subsystem3 ==
  In1 : Inport
  Enable : EnablePort
  CAN Transmit7 : canlib/CAN Transmit  BlockHandle=1293.0001  Device=MathWorks Virtual 1 (Channel 1)  DeviceMenu=MathWorks Virtual 1 (Channel 1)  ObjConstructor=canChannel('MathWorks', 'Virtual 1', 1)  EnableEventTransmit=off  EnablePeriodicTransmit=on  MessagePeriod=0.840
  wires:
  In1/1 -> CAN Transmit7/1

== system can-signal-sim/Subsystem4 ==
  In1 : Inport
  Enable : EnablePort
  CAN Transmit4 : canlib/CAN Transmit  BlockHandle=1302.0001  Device=MathWorks Virtual 1 (Channel 1)  DeviceMenu=MathWorks Virtual 1 (Channel 1)  ObjConstructor=canChannel('MathWorks', 'Virtual 1', 1)  EnableEventTransmit=off  EnablePeriodicTransmit=on  MessagePeriod=0.640
  wires:
  In1/1 -> CAN Transmit4/1

== system can-signal-sim/Subsystem9 ==
  In1 : Inport
  Enable : EnablePort
  CAN Transmit2 : canlib/CAN Transmit  BlockHandle=1311.0001  Device=MathWorks Virtual 1 (Channel 1)  DeviceMenu=MathWorks Virtual 1 (Channel 1)  ObjConstructor=canChannel('MathWorks', 'Virtual 1', 1)  EnableEventTransmit=off  EnablePeriodicTransmit=on  MessagePeriod=0.100
  wires:
  In1/1 -> CAN Transmit2/1

== system can-signal-sim/untitledPanel ==
  CTR_SISP_PO_GRB : ComboBox  Tag=HiddenForWebPanel  PanelInfo="{\"height\":25,\"left\":18,\"panelId\":\"panelId-b7a8a067-5a14-4b83-bf81-0b77a083025f\",\"top\":18,\"type\":\"panelChild\",\"version\":\"2019b\",\"width\":160,\"zIndex\":1500002}"  LabelPosition=Hide  SelectedLabel=aus
      settings: Values={{'aus', 'P', 'R', 'P_30sec', 'N', 'N30,5min', 'N_5min', 'D', 'Signal ungueltig'}, [0 1 2 3 4 6 7 8 15]}
  CTR_SISP_PO_GRB_COMP : ComboBox  Tag=HiddenForWebPanel  PanelInfo="{\"height\":25,\"left\":18,\"panelId\":\"panelId-b7a8a067-5a14-4b83-bf81-0b77a083025f\",\"top\":123,\"type\":\"panelChild\",\"version\":\"2019b\",\"width\":160,\"zIndex\":1500006}"  LabelPosition=Hide  SelectedLabel=Signal ungueltig
      settings: Values={{'aus', 'P', 'R', 'P_30sec', 'N', 'N30,5min', 'N_5min', 'D', 'Signal ungueltig'}, [15 14 13 12 11 9 8 7 0]}
  Combo Box : ComboBox  Tag=HiddenForWebPanel  PanelInfo="{\"height\":25,\"left\":18,\"panelId\":\"panelId-b7a8a067-5a14-4b83-bf81-0b77a083025f\",\"top\":228,\"type\":\"panelChild\",\"version\":\"2019b\",\"width\":160,\"zIndex\":1500004}"  LabelPosition=Hide  SelectedLabel=Dunkelschaltung
      settings: Values={{'Dunkelschaltung', '1.Gang', '2.Gang', '3.Gang', '4.Gang', '5.Gang', '6.Gang', '7.Gang', '8.Gang', 'Signal ungültig'}, [0 5 6 7 8 9 10 11 12 15]}
  Combo Box1 : ComboBox  Tag=HiddenForWebPanel  PanelInfo="{\"height\":25,\"left\":18,\"panelId\":\"panelId-b7a8a067-5a14-4b83-bf81-0b77a083025f\",\"top\":308,\"type\":\"panelChild\",\"version\":\"2019b\",\"width\":160,\"zIndex\":1500008}"  LabelPosition=Hide
      settings: Values={{'Label1', 'Label2', 'Label3'}, [0 1 2]}
  panelInfo : PanelWebBlock  Tag=HiddenForWebPanel  PanelInfo="{\"compacted\":false,\"height\":355,\"isActiveTab\":true,\"left\":406,\"name\":\"Panel\",\"panelId\":\"panelId-b7a8a067-5a14-4b83-bf81-0b77a083025f\",\"popoutData\":{\"height\":0,\"left\":0,\"maximized\":false,\"top\":0,\"width\":0},\"popoutMode\":\"componentHidden\",\"tabIndex\":0,\"tabbedSetId\":\"tabbedSet7917689624\",\"top\":237,\"type\":\"panel\",\"version\":\"2019b\",\"visible\":true,\"width\":200,\"zIndex\":1500002}"  PanelSnapshot=<binary blob, 20584 chars, not shown>

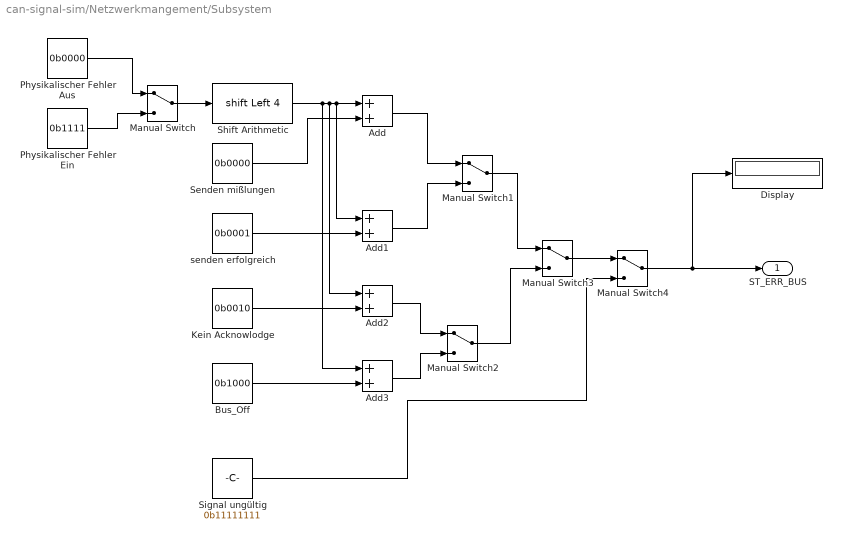
== system can-signal-sim/Netzwerkmangement/Subsystem ==
  Add{,1..3} (4 alike) : Sum
  Bus_Off : Constant  Value=0b1000
  Display : Display
      settings: Format=binary (Stored Integer)
  Kein Acknowlodge : Constant  Value=0b0010
  Manual Switch{,1..4} (5 alike) : ManualSwitch
  Physikalischer Fehler Aus : Constant  Value=0b0000
  Physikalischer Fehler Ein : Constant  Value=0b1111
  Senden mißlungen : Constant  Value=0b0000
  Shift Arithmetic : ArithShift  BitShiftNumber=4  BitShiftDirection=Left
  Signal ungültig : Constant  Value=0b11111111
  senden erfolgreich : Constant  Value=0b0001
  ST_ERR_BUS : Outport
  wires:
  Add1/1 -> Manual Switch1/2
  Manual Switch4/1 -> ST_ERR_BUS/1, Display/1
  Physikalischer Fehler Aus/1 -> Manual Switch/1
  Kein Acknowlodge/1 -> Add2/2
  Physikalischer Fehler Ein/1 -> Manual Switch/2
  Add2/1 -> Manual Switch2/1
  Add3/1 -> Manual Switch2/2
  Shift Arithmetic/1 -> Add2/1, Add1/1, Add/1, Add3/1
  Bus_Off/1 -> Add3/2
  Manual Switch1/1 -> Manual Switch3/1
  Add/1 -> Manual Switch1/1
  Manual Switch/1 -> Shift Arithmetic/1
  Manual Switch3/1 -> Manual Switch4/1
  Senden mißlungen/1 -> Add/2
  Manual Switch2/1 -> Manual Switch3/2
  Signal ungültig/1 -> Manual Switch4/2
  senden erfolgreich/1 -> Add1/2

== system can-signal-sim/Netzwerkmangement/Subsystem1 ==
  Combo Box1 : ComboBox  LabelPosition=Hide  SelectedLabel=Kombi
      settings: Values={{'JBBF', 'ACSM,MRSZ', 'RDC', 'CTM,CVM_V', 'Kombi'}, [1152 1153 1184 1188 1248]}
  Constant : Constant  Value=1248  OutDataTypeStr=uint16
  Display : Display
      settings: Format=binary (Stored Integer)
  Extract Bits : simulink/Logic and Bit Operations/Extract Bits  bitsToExtract=Range ending with least significant bit  numBits=7  bitIdxRange=[0 7]  outScalingMode=Preserve fixed-point scaling
  Irgendeine Adresse : Constant  Value=65
  Manual Switch : ManualSwitch
  RCVR : Outport
  wires:
  Constant/1 -> Extract Bits/1
  Extract Bits/1 -> Manual Switch/1
  Manual Switch/1 -> Display/1, RCVR/1
  Irgendeine Adresse/1 -> Manual Switch/2

== matlab function can-signal-sim/Bedienung Uhrzeit/MATLAB Function ==
  data: day output; month output; year output; isSummerTime output; hours output; minutes output; seconds output
function [day, month, year, isSummerTime, hours, minutes, seconds] = getTime()

    % Hole die aktuelle Systemzeit als Vektor
    timeVec = clock;  

    % Extrahiere Zeit- und Datumswerte
    year = timeVec(1);
    month = timeVec(2);
    day = timeVec(3);
    hours = timeVec(4);
    minutes = timeVec(5);
    seconds = floor(timeVec(6)); % Ganze Sekunden  

    % Berechne Sommerzeit (März - Oktober)
    if (month >= 3 && month <= 10)
        isSummerTime = true;
    else
        isSummerTime = false;
    end
end
